simulink model "Control_Logic_For_STM32"  (R2025b)
settings: Solver=VariableStepAuto  StartTime=0.0  StopTime=inf  FixedStep=1e-7  MaxStep=1/80000  RelTol=1e-3  EnableMultiTasking=on
model workspace (MAT data in the model file):
  Ki_ext = 0.1
  Kp_ext = 0.001
  Ref_I_ess_cmd = timeseries
  Ref_I_ess_cmd.Name = 'unnamed'
  Ref_I_ess_cmd.DataInfo = tsdata.datametadata
  Ref_I_ess_cmd.DataInfo.Interpolation = tsdata.interpolation
  Ref_I_ess_cmd.DataInfo.Interpolation.Fhandle : function handle (value not decoded)
  Ref_I_ess_cmd.DataInfo.Interpolation.Name = 'linear'
  Ref_I_ess_cmd.TimeInfo = tsdata.timemetadata
  Ref_I_ess_cmd.TimeInfo.Length = 6
  Ref_I_ess_cmd.TimeInfo.DuplicateTimes = 0
  Ref_I_ess_cmd.TimeInfo.Time_ = [0; 0.029999; 0.03; 0.059999; 0.06; 0.1]
  Ref_I_ess_cmd.TimeInfo.Initialized = 1
  Ref_I_ess_cmd.QualityInfo = tsdata.qualmetadata
  Ref_I_ess_cmd.Data_ = [10; 10; -10; -10; 10; 10]
  Ref_Ki_ext = timeseries
  Ref_Ki_ext.Name = 'unnamed'
  Ref_Ki_ext.DataInfo = tsdata.datametadata
  Ref_Ki_ext.DataInfo.Interpolation = tsdata.interpolation
  Ref_Ki_ext.DataInfo.Interpolation.Fhandle : function handle (value not decoded)
  Ref_Ki_ext.DataInfo.Interpolation.Name = 'linear'
  Ref_Ki_ext.TimeInfo = tsdata.timemetadata
  Ref_Ki_ext.TimeInfo.Length = 2
  Ref_Ki_ext.TimeInfo.DuplicateTimes = 0
  Ref_Ki_ext.TimeInfo.Time_ = [-1; 1.1]
  Ref_Ki_ext.TimeInfo.Initialized = 1
  Ref_Ki_ext.QualityInfo = tsdata.qualmetadata
  Ref_Ki_ext.Data_ = reshape([0.1 0.1], [1 1 2])
  Ref_Kp_ext = timeseries
  Ref_Kp_ext.Name = 'unnamed'
  Ref_Kp_ext.DataInfo = tsdata.datametadata
  Ref_Kp_ext.DataInfo.Interpolation = tsdata.interpolation
  Ref_Kp_ext.DataInfo.Interpolation.Fhandle : function handle (value not decoded)
  Ref_Kp_ext.DataInfo.Interpolation.Name = 'linear'
  Ref_Kp_ext.TimeInfo = tsdata.timemetadata
  Ref_Kp_ext.TimeInfo.Length = 2
  Ref_Kp_ext.TimeInfo.DuplicateTimes = 0
  Ref_Kp_ext.TimeInfo.Time_ = [-1; 1.1]
  Ref_Kp_ext.TimeInfo.Initialized = 1
  Ref_Kp_ext.QualityInfo = tsdata.qualmetadata
  Ref_Kp_ext.Data_ = reshape([0.001 0.001], [1 1 2])
  Ref_VH = timeseries
  Ref_VH.Name = 'unnamed'
  Ref_VH.DataInfo = tsdata.datametadata
  Ref_VH.DataInfo.Interpolation = tsdata.interpolation
  Ref_VH.DataInfo.Interpolation.Fhandle : function handle (value not decoded)
  Ref_VH.DataInfo.Interpolation.Name = 'linear'
  Ref_VH.TimeInfo = tsdata.timemetadata
  Ref_VH.TimeInfo.Length = 2
  Ref_VH.TimeInfo.DuplicateTimes = 0
  Ref_VH.TimeInfo.Time_ = [-1; 1.1]
  Ref_VH.TimeInfo.Initialized = 1
  Ref_VH.QualityInfo = tsdata.qualmetadata
  Ref_VH.Data_ = reshape([380 380], [1 1 2])
  SampleTime = Simulink.Parameter
  SampleTime.Value = 1e-07
  SampleTime.Complexity = 'real'
  SampleTime.Dimensions = [1 1]
  SampleTime.DataType = 'auto'
  V_batt = 96
  V_init_LV = 96
libraries: fl_lib x21, nesl_utility x21, ee_lib x8
settings Model: SILPILSystemUnderTest=refmodels  CodeVerificationMode=processor-in-the-loop (pil)  Creator=vivid  LastModifiedBy=vivid
settings OptimizationCC: DefaultParameterBehavior=Inlined  EnhancedBackFolding=on  PassReuseOutputArgsAs=Individual arguments  ZeroExternalMemoryAtStartup=off  ZeroInternalMemoryAtStartup=off  MaxStackSize=512  OptimizeBlockOrder=speed  DifferentSizesBufferReuse=on  OptimizationCustomize=off  EfficientTunableParamExpr=on
settings DebuggingCC: ParameterTunabilityLossMsg=error
settings HardwareCC: ProdBitPerPointer=32.0  ProdBitPerSizeT=32.0  ProdBitPerPtrDiffT=32.0  ProdLargestAtomicInteger=Long  ProdLargestAtomicFloat=Double  ProdWordSize=32.0  ProdLongLongMode=on  ProdHWDeviceType=ARM Compatible->ARM Cortex-M
settings SFSimCC: MATLABDynamicMemAlloc=off
settings RTWCC: SystemTargetFile=ert.tlc  HardwareBoard=STM32G4xx Based  TemplateMakefile=ert_default_tmf  Toolchain=GNU Tools for ARM Embedded Processors  Description=Embedded Coder
settings CodeAppCC: ForceParamTrailComments=on  IgnoreCustomStorageClasses=off  OperatorAnnotations=on  SimulinkDataObjDesc=on  SFDataObjDesc=on  InsertBlockDesc=on
settings ERTTargetCC: ExtModeTransport=3.0  ExtModeStaticAlloc=on  ExtModeStaticAllocSize=2048.0  ExtModeMexFile=ext_xcp  ExtModeIntrfLevel=Level2 - Open  RootIOFormat=Structure reference  TargetLangStandard=C99 (ISO)  CodeReplacementLibrary=ARM Cortex-M

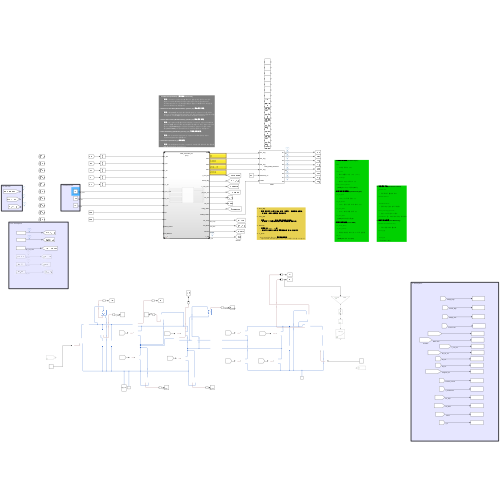
[thumbnail: Simulink's stored preview of the top-level diagram]
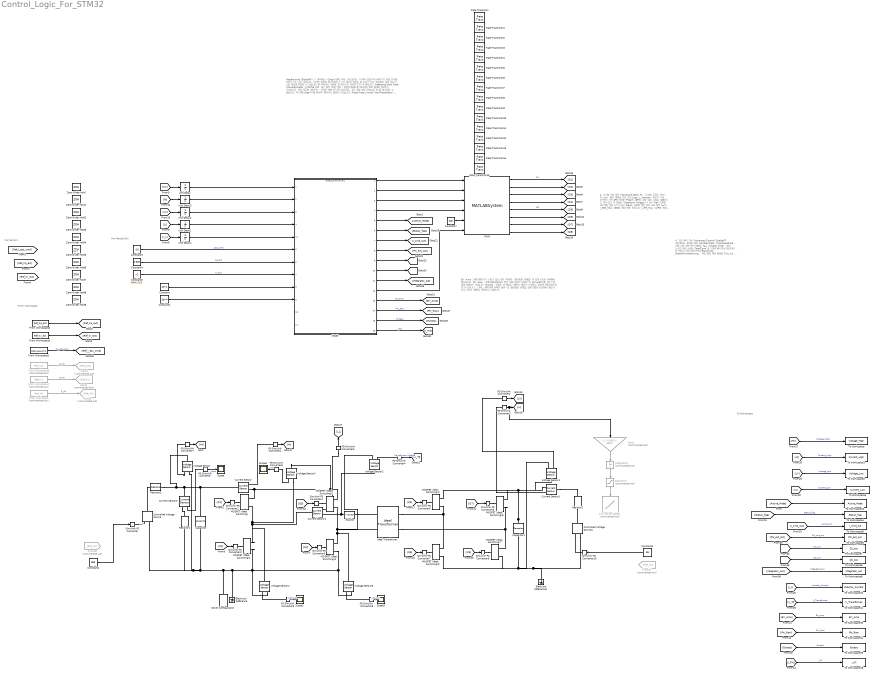
== system Control_Logic_For_STM32 ==
  note: 1e-7
  note: Feedforward (EnableFF) : [꺼주세요 / Check Off] 이유 : 피드포워드가 켜져 있으면 PI 제어기가 일을 안 해도 전류가 어느 정도 맞습니다. 이러면 최적화 알고리즘이 *"어? 게인이 작아도 잘 되네?"*라고 착각해서 반응 속도가 느린 게인을 추천할 수 있습니다. PI 혼자서도 외란을 잘 버티는지 보려면 끄는 게 좋습니다.
      |
      | Reference Slew Rate (MaxSlewRate) : [Infinite (inf) 또는 매우 크게] 이유 : 지령치(10A)를 부드럽게 램프 형태로 넣어주는 기능입니다. 이걸 켜두면 제어기는 "급격한 변화"를 겪지 않으므로, 과도 응답 성능(오버슈트 등)을 테스트할 수 없습니다. **"진짜 Step"**을 맞아야 제어기의 실력이 드러납니다.
      |
      | Phase Rate Limiter (MaxPhaseRate) : [Infinite (inf) 또는 매우 크게] 이유 : 위상각 변화 속도를 물리적으로 제한하는 기능입니다. 이걸 너무 빡빡하게 걸어두면, Kp를 아무리 키워도 반응이 빨라지지 않습니다. 또한, 게인이 너무 커서 생기는 진동(Oscillation)을 이 리미터가 숨겨버릴 수 있습니다. 진동은 **비용 함수(Control Effort)**가 잡아내도록 하고, 리미터는 풀어주는 게 좋습니다.
      |
      | Gain Scheduling (GainSched_Factor) : [1.0 (기본값)으로 설정] 이유 : 에러 크기에 따라 게인을 바꾸는 기능입니다. 최적화 중에는 게인이 고정되어야 결과 분석이 명확합니다.
      |
      | Dead Zone (DeadZone) : [0으로 설정] 이유 : 작은 에러를 0으로 무시하는 기능입니다. 미세한 잔류 편차까지 잡는 정밀한 Ki를 찾으려면 0으로 두어야 합니다.
  note: 4. 고급 제어 기능 (Advanced Control)
      | EnableFF
      | : 피드포워드 활성화 여부
      | MaxSlewRate
      | ,
      | MaxPhaseRate
      | : 전류/위상 급변 방지 제한값
      | Tau_Voltage_Filter
      | : 센싱 노이즈 필터 시정수
      | DeadZone 등: 미세 제어 튜닝 파라미터
      | 5. 변압기 자속 평형 (Flux Balancing)
      | EnableFluxBalancing
      | : 자속 평형 제어 활성화
      | Flux_Kp
      | ,
      | Flux_Ki
      | : 자속 제어기 게인
  note: 1. 시스템 기본 설정 (Hardware Spec)
      | Fs
      | : 스위칭 주파수 (Hz)
      | Ts_ctrl
      | : 제어 샘플링 시간 (Ts) [sec]
      | L_leakage
      | : 변압기 누설 인덕턴스 (H)
      | SPS_Inner_Phase
      | : [SPS] 내부 위상 고정값 (180도)
      | 2. 운전 모드 및 목표값 (Operation Targets)
      | V_HV_Ref
      | : [UPS] HV 목표 전압 (V)
      | V_HV_Band
      | : [UPS] 정전 감지 오차 범위 (±V)
      | I_ESS_Max
      | : [ESS] 최대 허용 전류 (A)
      | I_UPS_Max
      | : [UPS] 최대 허용 전류 (A)
      | 3. 배터리 보호 설정 (Smart BMS)
      | V_Pack_Max ~
      | V_Min_Limit
      | : 과충전/과방전 보호 및 CV 모드 설정값
      | K_CV
      | : [BMS] CV 제어 게인 (A/V)
  note: From Workspace
  note: To Workspace
  note: For Manual Sim
  note: For GA Sim
  note: Err_Amp
      | : 현재 제어기가 느끼고 있는 오차 (지령치 - 필터링된 실제값)
      | 이 값이 0으로 수렴해야 정상입니다.
      | Phi_Raw
      | : 포화(Saturation) 전의 원래 계산된 위상값
      | 이 값이 ±90도를 넘어가면 포화 상태라는 뜻입니다.
      | Excess
      | : 포화된 양 (Raw - 90도)
      | 제어기가 얼마나 심하게 포화되었는지 알 수 있습니다.
      | I_Filt
      | : 제어기에 실제로 들어가는 필터링된 전류값
      | 실제 전류와 비교해서 필터가 너무 느린지, 빠른지 판단할 수 있습니다.
  1-D Lookup Table2 : Lookup_n-D  Commented=on  NumberOfTableDimensions=1  BreakpointsForDimension1=[0, 0.1, 0.2, 0.3, 0.4, 0.5, 0.6, 0.7, 0.8, 0.9, 1.0]  Table=[84.0, 90.0, 93.0, 94.4, 95.6, 96.6, 98.0, 100.2, 103.0, 106.4, 109.2]  InternalRulePriority=Speed  RndMeth=Simplest
  Capacitor : fl_lib/Electrical/Electrical Elements/Capacitor  c=1000e-6 F  r=0.5 Ohm  g=0 1/Ohm  i_specify=off  i_priority=None  i=0 A  i_nominal_specify=off  i_nominal_value=1  i_nominal_unit=A  v_specify=on  v_priority=None  v=380 V  v_nominal_specify=off  v_nominal_value=1  v_nominal_unit=V  vc_specify=on  vc_priority=High  vc=380 V  vc_nominal_specify=off  vc_nominal_value=1  vc_nominal_unit=V
  Capacitor1 : fl_lib/Electrical/Electrical Elements/Capacitor  c=4700e-6 F  r=0.5 Ohm  g=0 1/Ohm  i_specify=off  i_priority=None  i=0 A  i_nominal_specify=off  i_nominal_value=1  i_nominal_unit=A  v_specify=on  v_priority=None  v=96 V  v_nominal_specify=off  v_nominal_value=1  v_nominal_unit=V  vc_specify=on  vc_priority=High  vc=96 V  vc_nominal_specify=off  vc_nominal_value=1  vc_nominal_unit=V
  Constant : Constant  Value=1e+1
  Constant1 : Constant  Value=1e+4
  Constant2 : Constant  Value=380
  Constant3 : Constant  Value=-10
  Constant4 : Constant  Value=2.625
  Constant5 : Constant  Value=96
  Constant6 : Constant  Value=49642.925
  Constant7 : Constant  Value=200
  Controlled Voltage Source : fl_lib/Electrical/Electrical Sources/Controlled Voltage Source
  Controlled Voltage Source1 : fl_lib/Electrical/Electrical Sources/Controlled Voltage Source
  Current Sensor{,1..3} (4 alike) : fl_lib/Electrical/Electrical Sensors/Current Sensor
  Electrical Reference : fl_lib/Electrical/Electrical Elements/Electrical Reference
  Electrical Reference1 : fl_lib/Electrical/Electrical Elements/Electrical Reference
  From Workspace : FromWorkspace  Commented=on  VariableName=Ref_VH
  From Workspace2 : FromWorkspace  VariableName=Ref_I_ess_cmd
  From Workspace4 : FromWorkspace  VariableName=Ref_Kp_ext
  From Workspace5 : FromWorkspace  VariableName=Ref_Ki_ext
  From Workspace6 : FromWorkspace  Commented=on  VariableName=Ref_Kpv
  From Workspace7 : FromWorkspace  Commented=on  VariableName=Ref_Kiv
  From37 : From  Commented=on  GotoTag=Ref_VL
  From38 : From  Commented=on  GotoTag=Ref_VH
  Gain2 : Gain  Commented=on  Gain=-1 / (0.0001 * 3600)
  Goto28 : Goto  Commented=on  GotoTag=Ref_VH
  Goto4 : Goto  Commented=on  GotoTag=Ref_Kpv
  Goto9 : Goto  Commented=on  GotoTag=Ref_Kiv
  Ideal Transformer : fl_lib/Electrical/Electrical Elements/Ideal Transformer  n=4  i1_specify=off  i1_priority=None  i1=0 A  i1_nominal_specify=off  i1_nominal_value=1  i1_nominal_unit=A  v1_specify=off  v1_priority=None  v1=0 V  v1_nominal_specify=off  v1_nominal_value=1  v1_nominal_unit=V  i2_specify=off  i2_priority=None  i2=0 A  i2_nominal_specify=off  i2_nominal_value=1  i2_nominal_unit=A  v2_specify=off  v2_priority=None  v2=0 V  v2_nominal_specify=off  v2_nominal_value=1  v2_nominal_unit=V
  Inductor : fl_lib/Electrical/Electrical Elements/Inductor  l=90e-6 H  r=0 Ohm  g=1e-9 1/Ohm  i_specify=off  i_priority=None  i=0 A  i_nominal_specify=off  i_nominal_value=1  i_nominal_unit=A  v_specify=off  v_priority=None  v=0 V  v_nominal_specify=off  v_nominal_value=1  v_nominal_unit=V  i_L_specify=off  i_L_priority=High  i_L=0 A  i_L_nominal_specify=off  i_L_nominal_value=1  i_L_nominal_unit=A
  Integrator2 : Integrator  Commented=on  InitialCondition=0.5
  MOSFET (Ideal, Switching){,1..7} (8 alike) : ee_lib/Semiconductors & Converters/MOSFET (Ideal, Switching)  port_option=ee.enum.controlport.ps  Rds=0.1 Ohm  Goff=1e-8 1/Ohm  Vth=2.7 V  diode_param=ee.enum.semiconductors.protectionDiode.nodynamics  diode_Vf=3.2 V  diode_Ron=0.1 Ohm  diode_Goff=1e-5 1/Ohm  diode_C=50e-9 F  diode_iRM=-235 A  diode_iF=300 A  diode_idot=-50 A/us  diode_trr_param=ee.enum.converters.diodeReverseParam.trr_factor  diode_trr_factor=3  diode_trr=15 us  diode_Qrr=1500 s*uA  ids_specify=off  ids_priority=None  ids=0 A  ids_nominal_specify=off  ids_nominal_value=1  ids_nominal_unit=A  vds_specify=off  vds_priority=None  vds=0 V  vds_nominal_specify=off  vds_nominal_value=1  vds_nominal_unit=V  vgs_specify=off  vgs_priority=None  vgs=0 V  vgs_nominal_specify=off  vgs_nominal_value=1  vgs_nominal_unit=V  thermal_loss_option=ee.enum.converters.thermalLossOption.constantvalues  Von_data=[0, 1.8, 3.2, 6, 10, 16; 0, 2, 5.5, 9.5, 15, 25] V  Tj=[298.15, 448.15] K  Iout_data=[0, 20, 40, 60, 80, 100] A  Eon_data=[0, 55.04, 124.57, 235.53, 362.12; 0, 71.25, 161.25, 304.88, 468.75] * 1e-6 J  Eoff_data=[0, 18, 30, 56.1, 76.5; 0, 22.5, 37.5, 70.13, 95.63] * 1e-6 J  Eon_data_3D=[zeros(2, 5, 3)] J  Eoff_data_3D=[zeros(2, 5, 3)] J  Tj_loss=[298.15, 448.15] K  Iout_data_loss=[0, 10, 20, 30, 40] A  tabulateWithVds=false  Vds_loss=[0, 150, 300] V  Eon_scalar=22.86e-3 J  Eoff_scalar=17.14e-3 J  Voff=300 V  Iout_scalar=600 A  useCurrentFromPreviousCycle=false  useVoltageFromPreviousCycle=false  diodeModelType=ee.enum.converters.diodeModelType.pwl  diodeTableType=ee.enum.diode.tableType.IfMat  diode_ReverseIVType=ee.enum.diode.diodeReverseIV.constant  diode_IfMat=[.07, .12, .19, 1.75, 4.24, 7.32, 11.2; .16, .3, .72, 2.14, 4.02, 6.35, 9.12] A  diode_VfMat=[.9, 1.15, 1.25, 1.5, 1.75, 2.17, 2.6, 2.85; .58, .68, .75, 1.1, 1.38, 1.77, 2.27, 2.7] V  diode_TjVec=[25, 125] degC  diode_VfVec=[.5, .7, .9, 1.3, 1.7, 2.1, 2.5] V  diode_IfVec=[.1, .2, .5, 1, 2, 4, 7, 10] A  diode_IrMat=[1e-06, 2e-06, 5e-06, 1e-05, 2.5e-05, 5e-05, .0001; 2e-06, 5e-06, 1e-05, 4e-05, 8e-05, .0002, .0005] A  diode_VrMat=[10, 100, 200, 250, 300, 325, 350; 10, 70, 160, 220, 270, 300, 320] V  diode_VrVec=[10, 20, 40, 50, 70, 80, 100] V  diode_IrVec=[1e-06, 2e-06, 5e-06, 1e-05, 2e-05, 5e-05, .0001] A  diode_Vr=-600 V  diode_Ls=150 nH  diode_Erec=0.03 J  diode_rec_loss_model=ee.enum.diode.reverseRecoveryModel.fixed  diode_ErecVal=0 J  diode_scaleWithIandV=true  diode_ErecMat=zeros(2, 3) J  diode_TjrecVec=[298.15, 398.15] K  diode_IfrecVec=[.1, 1, 10] A  diode_IrecVal=10 A  diode_VrecVal=10 V  diode_tFilter=1 / 1000 / 100 s  separateThermalPortForDiode=false  thermal_network_parameterization=ee.enum.thermalNetworkTopology.external  Rth=[.03, .2] K/W  Rth_Cauer=[.03, .1, .2] K/W  Rth_Foster=[.08, .14, .22, .16] K/W  thermal_mass_parameterization=ee.enum.thermalNetwork.timeconstant  thermal_mass=[3, 25] J/K  thermal_mass_Cauer=[3, 10, 25] J/K  thermal_mass_Foster=[.001, .005, .05, .5] J/K  thermal_time_constant=[.1, 5] s  thermal_time_constant_Cauer=[.1, 1, 5] s  thermal_time_constant_Foster=[7e-05, .0007, .01, .08] s  thermal_mass_initial_temperatures=[25, 25] degC  thermal_mass_initial_temperatures_Cauer=[25, 25, 25] degC  junction_thermal_mass=0.1 J/K  Tvec_initial_Foster=[25, 25, 25, 25] degC  RthDiode=[.03, .2] K/W  RthCauerDiode=[.03, .1, .2] K/W  RthFosterDiode=[.03, .2] K/W  thermalMassDiode=[3, 25] J/K  thermalMassCauerDiode=[3, 10, 25] J/K  thermalMassFosterDiode=[33, 50] J/K  thermalTauDiode=[.1, 5] s  thermalTauCauerDiode=[.1, 1, 5] s  thermalTauFosterDiode=[1, 10] s  thermalMassInitTempDiode=[25, 25] degC  thermalMassInitTempCauerDiode=[25, 25, 25] degC  junctionthermalMassDiode=0.1 J/K  TVecInitialFosterDiode=[25, 25, 25, 25] degC  no_thermal_network=0  mosfet_junction_temperature_specify=off  mosfet_junction_temperature_priority=None  mosfet_junction_temperature=25 degC  mosfet_junction_temperature_nominal_specify=off  mosfet_junction_temperature_nominal_value=1  mosfet_junction_temperature_nominal_unit=degC  diode_junction_temperature_specify=off  diode_junction_temperature_priority=None  diode_junction_temperature=25 degC  diode_junction_temperature_nominal_specify=off  diode_junction_temperature_nominal_value=1  diode_junction_temperature_nominal_unit=degC  Qj_specify=off  Qj_priority=None  Qj=0 W  Qj_nominal_specify=off  Qj_nominal_value=1  Qj_nominal_unit=W  accumulatedSwitchingLosses_specify=off  accumulatedSwitchingLosses_priority=None  accumulatedSwitchingLosses=0 J
  Model : ModelReference  ModelNameDialog=DAB_Controller_PIL.slx  SimulationMode=Processor-in-the-loop (PIL)  ModelReferenceVersion=1.66
      settings: PortSchema="{\"entries\":[{\"content\":{\"sides\":[{\"content\":{\"connectorIds\":[\"In1\",\"In2\",\"In3\",\"In4\",\"In12\",\"In5\",\"In6\",\"In7\",\"In8\",\"In9\",\"In10\",\"In11\"]},\"type\":\"ConnectorPlacement.EquallySpacedRectSide\",\"uuid\":\"fa4bbdd1-d2e9-4e1e-9678-f869006e0555\"},{\"content\":{\"connectorIds\":[\"Out1\",\"Out2\",\"Out3\",\"Out4\",\"Out5\",\"Out6\",\"Out7\",\"Out8\",\"Out9\",\"Out10\",\"Out11\",\"Out12\",\"Out13\",\"Out14\",\"Out15\",\"Out16\"],\"side\":\"RIGHT\"},\"type\":\"ConnectorPlacement.EquallySpacedRectSide\",\"uuid\":\"1ce66cfc-7a63-4184-ae37-29813a20eac6\"},{\"content\":{\"side\":\"TOP\"},\"type\":\"ConnectorPlacement.EquallySpacedRectSide\",\"uuid\":\"e125aaf4-3c4e-47ae-bf7a-f1e82defe1dc\"}]},\"type\":\"ConnectorPlacement.EquallySpacedConnector\",\"uuid\":\"4f71e27b-5f94-4311-80ee-f62e7bcdf7cb\"}],\"packageUris\":[\"http://schema.mathworks.com/mf0/Connector/R2020b\"],\"version\":\"1.0\"}"
  PS-Simulink Converter{,1..9} (10 alike) : nesl_utility/PS-Simulink Converter  PhysicalDomain=network_engine_domain  SubClassName=ps_output  LeftPortType=input  RightPortType=output  PseudoPeriodic=off  Frequencies=[]  VectorFormat=inherit  Unit=inherit  AffineConversion=off
  PWM : MATLABSystem  System=DAB_PWM_Generator  Fs=80e3  Ts_sim=1e-7  V_Gate_ON=18  V_Gate_OFF=-4  SimulateUsing=Code generation
      mask Type: DAB_PWM_Generator
  Rate Transition{,1..15} (16 alike) : RateTransition  OutPortSampleTime=SampleTime
  Resistor1 : fl_lib/Electrical/Electrical Elements/Resistor  R=100 Ohm  i_specify=off  i_priority=None  i=0 A  i_nominal_specify=off  i_nominal_value=1  i_nominal_unit=A  v_specify=on  v_priority=None  v=380 V  v_nominal_specify=off  v_nominal_value=1  v_nominal_unit=V
  Resistor2 : fl_lib/Electrical/Electrical Elements/Resistor  R=0.02 Ohm  i_specify=off  i_priority=None  i=0 A  i_nominal_specify=off  i_nominal_value=1  i_nominal_unit=A  v_specify=off  v_priority=None  v=0 V  v_nominal_specify=off  v_nominal_value=1  v_nominal_unit=V
  Resistor3 : fl_lib/Electrical/Electrical Elements/Resistor  R=0.01 Ohm  i_specify=off  i_priority=None  i=0 A  i_nominal_specify=off  i_nominal_value=1  i_nominal_unit=A  v_specify=off  v_priority=None  v=0 V  v_nominal_specify=off  v_nominal_value=1  v_nominal_unit=V
  Saturation : Saturate  Commented=on  UpperLimit=1  LowerLimit=0
  Scope{,1..3} (4 alike) : Scope
      Scope2 settings: DataLoggingVariableName=ScopeData2
      Scope3 settings: DataLoggingVariableName=ScopeData3
  Simulink-PS Converter{,2..10} (10 alike) : nesl_utility/Simulink-PS Converter  PhysicalDomain=network_engine_domain  SubClassName=ps_input  LeftPortType=input  RightPortType=output  PseudoPeriodic=off  Frequencies=[]  NoiseDistribution=none  NoiseParameters=[]  Unit=1  AffineConversion=off  FilteringAndDerivatives=provide  SimscapeFilterOrder=1  InputFilterTimeConstant=0.001  UdotUserProvided=0
  Solver Configuration : nesl_utility/Solver Configuration  PhysicalDomain=network_engine_domain  SubClassName=solver  LeftPortType=input  RightPortType=generic  Tones=[]  Harmonics=[]  SimulateNoise=off  Profile=off  UseLocalSampling=off  EnableSwitchedLinearOptims=on  FrequencyDomain=off  UseCCode=off  RelTol=0.001  AbsTol=0.001  MinStep=1e-09  ToWorkspace=off  RevertToSquareIcSolve=off  NumHomotopyIterations=100  PhasorMode=off  PhasorModeNumHarmonics=1  ConsistencySolver=NEWTON_XTOL_AFTER_FTOL  IndexReductionMethod=DerivativeReplacement  DoDC=off  ResidualTolerance=1e-09  ConsistencyTolSource=GLOBAL  ConsistencyAbsTol=0.001  ConsistencyRelTol=0.001  ConsistencyTolFactor=0.001  UseLocalSolver=off  LocalSolverChoice=NE_BACKWARD_EULER_ADVANCER  ResolveIndetEquations=on  FunctionEvalNumThread=1  LocalSolverSampleTime=0.001  DoFixedCost=off  MaxNonlinIter=3  MaxModeIter=2  ComputeImpulses=off  ImpulseIterations=2  LinearAlgebra=auto  LinearAlgebraNumThread=0  EquationFormulation=NE_TIME_EF  DelaysMemoryBudget=1024  AutomaticFiltering=off  FilteringTimeConstant=0.001  PartitionStorageMethod=AS_NEEDED  PartitionMemoryBudget=1024  PartitionMethod=ROBUST  MultibodyUseLocalSolver=off  MultibodyLocalSolverChoice=ODE1  MultibodyLocalSolverSampleTime=0.001
  To Workspace : ToWorkspace  VariableName=Voltage_High  SaveFormat=Timeseries  SampleTime=-1
  To Workspace1 : ToWorkspace  VariableName=Current_High  SaveFormat=Timeseries  SampleTime=-1
  To Workspace10 : ToWorkspace  VariableName=Inductor_Current  SaveFormat=Timeseries  SampleTime=-1
  To Workspace11 : ToWorkspace  VariableName=V_Transformer  SaveFormat=Timeseries  SampleTime=-1
  To Workspace12 : ToWorkspace  VariableName=Active_Mode  SaveFormat=Timeseries  SampleTime=-1
  To Workspace13 : ToWorkspace  VariableName=Err_Amp  SaveFormat=Timeseries  SampleTime=-1
  To Workspace14 : ToWorkspace  VariableName=Phi_Raw  SaveFormat=Timeseries  SampleTime=-1
  To Workspace15 : ToWorkspace  VariableName=Excess  SaveFormat=Timeseries  SampleTime=-1
  To Workspace16 : ToWorkspace  VariableName=I_Fil  SaveFormat=Timeseries  SampleTime=-1
  To Workspace2 : ToWorkspace  VariableName=Voltage_Low  SaveFormat=Timeseries  SampleTime=-1
  To Workspace3 : ToWorkspace  VariableName=Current_Low  SaveFormat=Timeseries  SampleTime=-1
  To Workspace4 : ToWorkspace  VariableName=Status_flag  SaveFormat=Timeseries  SampleTime=-1
  To Workspace5 : ToWorkspace  VariableName=I_cmd_out  SaveFormat=Timeseries  SampleTime=-1
  To Workspace6 : ToWorkspace  VariableName=Phi_ext_out  SaveFormat=Timeseries  SampleTime=-1
  To Workspace7 : ToWorkspace  VariableName=D1_out  SaveFormat=Timeseries  SampleTime=-1
  To Workspace8 : ToWorkspace  VariableName=D2_out  SaveFormat=Timeseries  SampleTime=-1
  To Workspace9 : ToWorkspace  VariableName=Integrator_out  SaveFormat=Timeseries  SampleTime=-1
  Unit Delay{,1..4} (5 alike) : UnitDelay  SampleTime=-1  HasFrameUpgradeWarning=on
  Voltage Sensor{,1..5} (6 alike) : fl_lib/Electrical/Electrical Sensors/Voltage Sensor
  Zero-Order Hold{,1..9} (10 alike) : ZeroOrderHold  SampleTime=SampleTime
  wires:
  [HV] -> Unit Delay/1
  [HI] -> Unit Delay3/1
  [LV] -> Unit Delay2/1
  [LI] -> Unit Delay1/1
  PS-Simulink Converter4/1 -> [V_Tf]  "Transformer Voltage"
  PS-Simulink Converter1/1 -> [HI]
  PS-Simulink Converter2/1 -> [LV]
  PS-Simulink Converter3/1 -> Gain2/1, [LI]
  PS-Simulink Converter5/1 -> [I_L]
  [Q1] -> Simulink-PS Converter2/1
  [Q4] -> Simulink-PS Converter5/1
  [Q2] -> Simulink-PS Converter3/1
  [Q3] -> Simulink-PS Converter4/1
  [Q5] -> Simulink-PS Converter6/1
  [Q6] -> Simulink-PS Converter7/1
  [Q8] -> Simulink-PS Converter8/1
  [Q7] -> Simulink-PS Converter9/1
  PS-Simulink Converter7/1 -> [HV]
  [I_L] -> To Workspace10/1  "Inductor_Current"
  [V_Tf] -> To Workspace11/1  "V_Transformer"
  [HV] -> To Workspace/1  "Voltage_High"
  [HI] -> To Workspace1/1  "Current_High"
  [LV] -> To Workspace2/1  "Voltage_Low"
  [LI] -> To Workspace3/1  "Current_Low"
  [Status_flag] -> To Workspace4/1  "Status_flag"
  [I_cmd_out] -> To Workspace5/1  "I_cmd_out"
  [Phi_ext_out] -> To Workspace6/1  "Phi_ext_out"
  [D1_out] -> To Workspace7/1  "D1_out"
  [D2_out] -> To Workspace8/1  "D2_out"
  [Integrator_out] -> To Workspace9/1  "Integrator_out"
  From Workspace2/1 -> [Ref_I_ess_cmd]  "R_I_ess_cmd"
  From Workspace/1 -> Goto28/1  "R_VH"
  PS-Simulink Converter/1 -> Scope/1  "I_Load"
  PWM/1 -> [Q1]  "D1"
  PWM/2 -> [Q2]
  PWM/5 -> [Q5]  "D5"
  PWM/6 -> [Q6]
  Constant7/1 -> PWM/5
  PS-Simulink Converter6/1 -> Scope1/1  "Vds"
  PS-Simulink Converter9/1 -> Scope2/1  "V_tf_high"
  PS-Simulink Converter8/1 -> Scope3/1  "V_tf_low"
  PWM/4 -> [Q4]
  PWM/3 -> [Q3]
  PWM/7 -> [Q7]
  PWM/8 -> [Q8]
  [Active_Mode] -> To Workspace12/1
  Gain2/1 -> Integrator2/1
  Constant5/1 -> Simulink-PS Converter10/1
  Constant2/1 -> Simulink-PS Converter/1
  Model/16 -> [I_Filt]  "I_Filt"
  Model/15 -> [Excess]  "Excess"
  Model/14 -> [Phi_Raw]  "Phi_Raw"
  Model/13 -> [Err_Amp]  "Err_Amp"
  From Workspace5/1 -> [Ref_Ki_ext]
  From Workspace4/1 -> [Ref_Kp_ext]
  From Workspace6/1 -> Goto4/1  "R_VH"
  From Workspace7/1 -> Goto9/1  "R_VH"
  Constant6/1 -> Model/7  "Ki_ext"
  Constant3/1 -> Model/5  "I_ess_cmd"
  Constant4/1 -> Model/6  "Kp_ext"
  Integrator2/1 -> Saturation/1
  Saturation/1 -> 1-D Lookup Table2/1
  [I_L] -> Unit Delay4/1
  [Err_Amp] -> To Workspace13/1  "Err_Amp"
  [Phi_Raw] -> To Workspace14/1  "Phi_Raw"
  [Excess] -> To Workspace15/1  "Excess"
  [I_Filt] -> To Workspace16/1  "I_Fil"
  Unit Delay/1 -> Model/1
  Unit Delay3/1 -> Model/2
  Unit Delay2/1 -> Model/3
  Unit Delay1/1 -> Model/4
  Unit Delay4/1 -> Model/12
  Constant/1 -> Model/8
  Constant1/1 -> Model/9
  Model/1 -> PWM/1
  Model/2 -> PWM/2
  Model/3 -> PWM/3
  Model/4 -> PWM/4
  Model/5 -> [Active_Mode]
  Model/6 -> [Status_flag]
  Model/7 -> [I_cmd_out]
  Model/8 -> [Phi_ext_out]
  Model/9 -> [D1_out]
  Model/10 -> [D2_out]
  Model/11 -> [Integrator_out]
  Model/12 -> PWM/6
  connections:
  Current Sensor/RConn2 -- "MOSFET (Ideal, Switching)"/RConn1 -- Voltage Sensor3/LConn1 -- "MOSFET (Ideal, Switching)2"/RConn1
  Ideal Transformer/RConn1 -- "MOSFET (Ideal, Switching)3"/RConn2 -- "MOSFET (Ideal, Switching)5"/RConn1
  Current Sensor2/LConn1 -- "MOSFET (Ideal, Switching)"/RConn2 -- Voltage Sensor3/RConn2 -- "MOSFET (Ideal, Switching)1"/RConn1 -- Voltage Sensor4/LConn1
  Inductor/RConn1 -- Ideal Transformer/LConn1
  "MOSFET (Ideal, Switching)4"/RConn1 -- Voltage Sensor2/RConn2 -- Ideal Transformer/LConn2 -- "MOSFET (Ideal, Switching)2"/RConn2 -- Voltage Sensor5/LConn1
  Capacitor1/LConn1 -- "MOSFET (Ideal, Switching)6"/RConn1 -- "MOSFET (Ideal, Switching)3"/RConn1 -- Voltage Sensor1/LConn1 -- Current Sensor1/RConn2
  "MOSFET (Ideal, Switching)1"/RConn2 -- "MOSFET (Ideal, Switching)4"/RConn2 -- Voltage Sensor5/RConn2 -- Voltage Sensor4/RConn2 -- Electrical Reference/LConn1 -- Controlled Voltage Source/RConn2 -- Resistor1/RConn1 -- Voltage Sensor/RConn2 -- Capacitor/RConn1 -- Solver Configuration/RConn1
  Capacitor1/RConn1 -- "MOSFET (Ideal, Switching)7"/RConn2 -- "MOSFET (Ideal, Switching)5"/RConn2 -- Voltage Sensor1/RConn2 -- Electrical Reference1/LConn1 -- Controlled Voltage Source1/RConn2
  "MOSFET (Ideal, Switching)6"/RConn2 -- Ideal Transformer/RConn2 -- "MOSFET (Ideal, Switching)7"/RConn1
  PS-Simulink Converter1/LConn1 -- Current Sensor/RConn1
  PS-Simulink Converter2/LConn1 -- Voltage Sensor1/RConn1
  PS-Simulink Converter3/LConn1 -- Current Sensor1/RConn1
  PS-Simulink Converter4/LConn1 -- Voltage Sensor2/RConn1
  Simulink-PS Converter/RConn1 -- Controlled Voltage Source/RConn1
  Inductor/LConn1 -- Voltage Sensor2/LConn1 -- Current Sensor2/RConn2
  PS-Simulink Converter5/LConn1 -- Current Sensor2/RConn1
  Simulink-PS Converter2/RConn1 -- "MOSFET (Ideal, Switching)"/LConn1
  Simulink-PS Converter3/RConn1 -- "MOSFET (Ideal, Switching)1"/LConn1
  Simulink-PS Converter4/RConn1 -- "MOSFET (Ideal, Switching)2"/LConn1
  Simulink-PS Converter5/RConn1 -- "MOSFET (Ideal, Switching)4"/LConn1
  Simulink-PS Converter6/RConn1 -- "MOSFET (Ideal, Switching)3"/LConn1
  Simulink-PS Converter7/RConn1 -- "MOSFET (Ideal, Switching)5"/LConn1
  Simulink-PS Converter8/RConn1 -- "MOSFET (Ideal, Switching)7"/LConn1
  Simulink-PS Converter9/RConn1 -- "MOSFET (Ideal, Switching)6"/LConn1
  Voltage Sensor/RConn1 -- PS-Simulink Converter7/LConn1
  Simulink-PS Converter10/RConn1 -- Controlled Voltage Source1/RConn1
  Current Sensor3/RConn2 -- Resistor1/LConn1
  PS-Simulink Converter/LConn1 -- Current Sensor3/RConn1
  PS-Simulink Converter6/LConn1 -- Voltage Sensor3/RConn1
  PS-Simulink Converter9/LConn1 -- Voltage Sensor4/RConn1
  PS-Simulink Converter8/LConn1 -- Voltage Sensor5/RConn1
  Current Sensor1/LConn1 -- Resistor2/LConn1
  Voltage Sensor/LConn1 -- Current Sensor/LConn1 -- Capacitor/LConn1 -- Current Sensor3/LConn1 -- Resistor3/RConn1
  Resistor3/LConn1 -- Controlled Voltage Source/LConn1
  Resistor2/RConn1 -- Controlled Voltage Source1/LConn1
